simulink model "ac_checks_A_test"  (R2018b)
settings: Solver=ode45  StartTime=0.0  StopTime=200  RelTol=1e-3
PreLoadFcn:
  | load_system('../simulink_reference_models/test_sequence_lib');
InitFcn:
  | close all
  | clear all
  | 
  | T_CNTL = 1/5e3;
  | 
  | VLL_NOM = 35e3;
  | F_NOM = 60;
libraries: test_sequence_lib x5
settings Model: SimulationMode=rapid-accelerator  Creator=HussamAlatrash  LastModifiedBy=ahhei
settings DataIOCC: ReturnWorkspaceOutputs=on
settings DebuggingCC: UnconnectedInputMsg=none  UnconnectedOutputMsg=none  UnconnectedLineMsg=none
settings ModelReferenceCC: EnableRefExpFcnMdlSchedulingChecks=off
settings RTWCC: Description=Generic Real-Time Target
settings ConfigComp: CovBoundaryAbsTol=1.0e-5

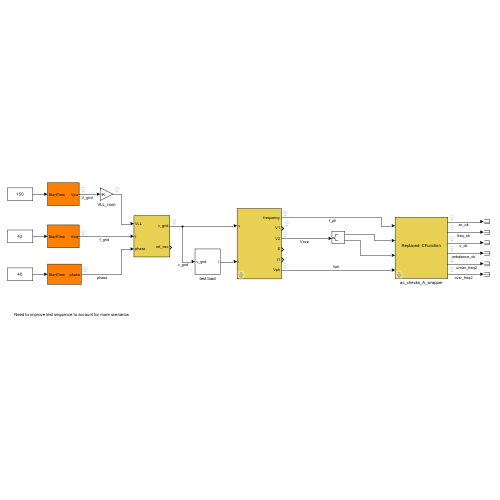
[thumbnail: Simulink's stored preview of the top-level diagram]
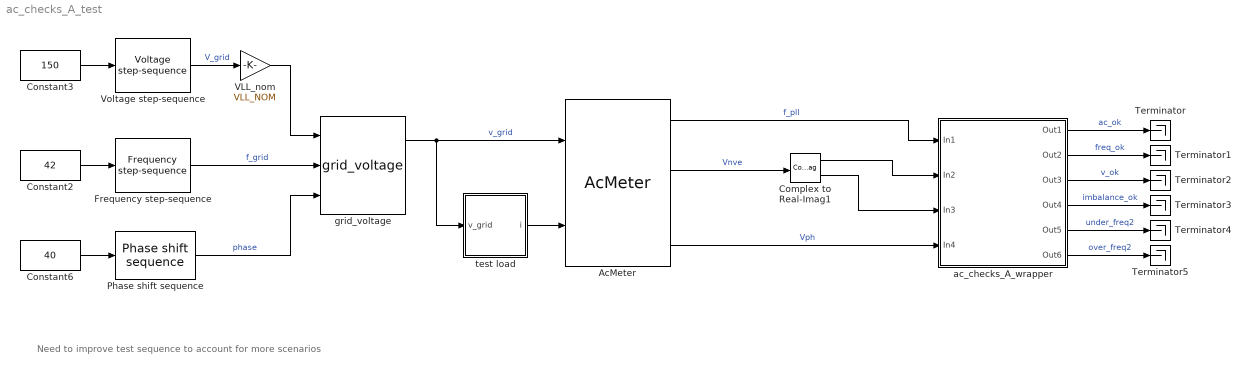
== system ac_checks_A_test ==
  note: Need to improve test sequence to account for more scenarios
  AcMeter : test_sequence_lib/AcMeter  VllRated=VLL_NOM
  Complex to Real-Imag1 : ComplexToRealImag
  Constant2 : Constant  Value=42
  Constant3 : Constant  Value=150
  Constant6 : Constant  Value=40
  Frequency step-sequence : test_sequence_lib/Frequency step-sequence  SystemSampleTime=-1  EmptyChoice=off  PassThrough=off  PassThroughVariantControl=(default)  EmptyChoiceVariantControl=(default)  Latency=0  AutoFrameSizeCalculation=off
  Phase shift sequence : test_sequence_lib/Phase shift sequence  SystemSampleTime=-1  EmptyChoice=off  PassThrough=off  PassThroughVariantControl=(default)  EmptyChoiceVariantControl=(default)  Latency=0  AutoFrameSizeCalculation=off
  Terminator{,1..5} (6 alike) : Terminator
  VLL_nom : Gain  Gain=VLL_NOM
  Voltage step-sequence : test_sequence_lib/Voltage step-sequence  SystemSampleTime=-1  EmptyChoice=off  PassThrough=off  PassThroughVariantControl=(default)  EmptyChoiceVariantControl=(default)  Latency=0  AutoFrameSizeCalculation=off
  ac_checks_A_wrapper : Subsystem  Description=Replaced Block  mask(Replaced Block){}
      mask help: This block has been replaced with an empty subsystem because it used functionality that is unavailable in Simulink R2018b.
      mask Display: fprintf('Replaced: %s\n','CFunction')
  grid_voltage : test_sequence_lib/grid_voltage  SystemSampleTime=-1  EmptyChoice=off  PassThrough=off  PassThroughVariantControl=(default)  EmptyChoiceVariantControl=(default)  Latency=0  AutoFrameSizeCalculation=off
  test load : Subsystem
  wires:
  VLL_nom/1 -> grid_voltage/1
  Phase shift sequence/1 -> grid_voltage/3  "phase"
  Voltage step-sequence/1 -> VLL_nom/1  "V_grid"
  Constant3/1 -> Voltage step-sequence/1
  Frequency step-sequence/1 -> grid_voltage/2  "f_grid"
  Constant2/1 -> Frequency step-sequence/1
  Constant6/1 -> Phase shift sequence/1
  grid_voltage/1 -> AcMeter/1, test load/1(v_grid)  "v_grid"
  test load/1(i) -> AcMeter/2
  AcMeter/1 -> ac_checks_A_wrapper/1(In1)  "f_pll"
  ac_checks_A_wrapper/2(Out2) -> Terminator1/1  "freq_ok"
  ac_checks_A_wrapper/1(Out1) -> Terminator/1  "ac_ok"
  ac_checks_A_wrapper/3(Out3) -> Terminator2/1  "v_ok"
  ac_checks_A_wrapper/4(Out4) -> Terminator3/1  "imbalance_ok"
  ac_checks_A_wrapper/5(Out5) -> Terminator4/1  "under_freq2"
  ac_checks_A_wrapper/6(Out6) -> Terminator5/1  "over_freq2"
  Complex to Real-Imag1/1 -> ac_checks_A_wrapper/2(In2)
  Complex to Real-Imag1/2 -> ac_checks_A_wrapper/3(In3)
  AcMeter/3 -> Complex to Real-Imag1/1  "Vnve"
  AcMeter/6 -> ac_checks_A_wrapper/4(In4)  "Vph"

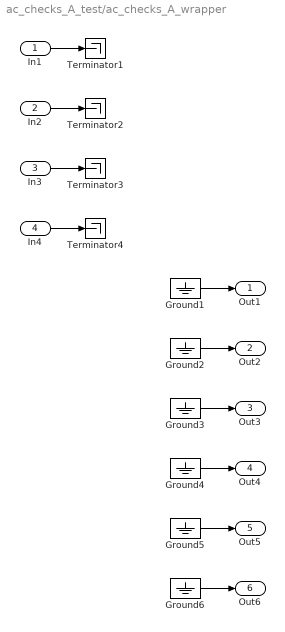
== system ac_checks_A_test/ac_checks_A_wrapper ==
  In1 : Inport
  In2 : Inport  Port=2
  In3 : Inport  Port=3
  In4 : Inport  Port=4
  Ground{1..6} (6 alike) : Ground
  Terminator{1..4} (4 alike) : Terminator
  Out1 : Outport
  Out2 : Outport  Port=2
  Out3 : Outport  Port=3
  Out4 : Outport  Port=4
  Out5 : Outport  Port=5
  Out6 : Outport  Port=6
  wires:
  Ground6/1 -> Out6/1
  Ground5/1 -> Out5/1
  Ground4/1 -> Out4/1
  Ground3/1 -> Out3/1
  Ground2/1 -> Out2/1
  Ground1/1 -> Out1/1
  In4/1 -> Terminator4/1
  In3/1 -> Terminator3/1
  In2/1 -> Terminator2/1
  In1/1 -> Terminator1/1

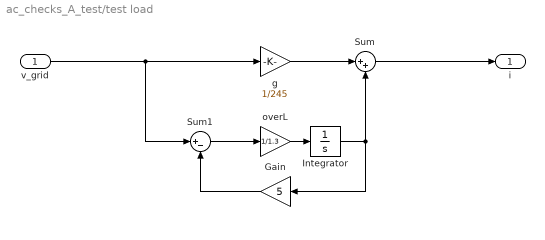
== system ac_checks_A_test/test load ==
  v_grid : Inport
  Gain : Gain  Gain=5
  Integrator : Integrator
  Sum : Sum  Inputs=|++
  Sum1 : Sum  Inputs=|+-
  g : Gain  Gain=1/245
  overL : Gain  Gain=1/1.3
  i : Outport
  wires:
  v_grid/1 -> g/1, Sum1/1
  overL/1 -> Integrator/1
  Integrator/1 -> Gain/1, Sum/2
  Sum1/1 -> overL/1
  Sum/1 -> i/1
  g/1 -> Sum/1
  Gain/1 -> Sum1/2
